simulink model "ARDroneHoverSim_backup_2026-11-11"  (R2025b)
settings: Solver=ode1  StartTime=0.0  StopTime=100  FixedStep=simDT  RelTol=1e-3  EnableMultiTasking=on
undefined symbols (not defined in the file or in its folder): FMS
libraries: ARBlocks x2
settings Model: Creator=Paul Freeman  LastModifiedBy=caio
settings SolverCC: AlgebraicLoopSolver=TrustRegion
settings DataIOCC: SaveFormat=Array  SignalLoggingSaveFormat=ModelDataLogs  SaveOutput=off  SignalLogging=off  ReturnWorkspaceOutputs=off
settings OptimizationCC: ExpressionDepthLimit=2147483647.0  LifeSpan=inf
settings DebuggingCC: UnderspecifiedInitializationDetection=Classic  MergeDetectMultiDrivingBlocksExec=none  SolverPrmCheckMsg=warning  MultiTaskDSMMsg=warning  MultiTaskCondExecSysMsg=none  FcnCallInpInsideContextMsg=warning  UnconnectedInputMsg=warning  UnconnectedOutputMsg=warning  UnconnectedLineMsg=warning  StateNameClashWarn=warning  SFUnexpectedBacktrackingDiag=warning  SFNoUnconditionalDefaultTransitionDiag=warning  SFExecutionAtInitializationDiag=none  ArithmeticOperatorsInVariantConditions=warning
settings HardwareCC: ProdBitPerPointer=32.0  ProdBitPerSizeT=32.0  ProdBitPerPtrDiffT=32.0  ProdLargestAtomicInteger=Long  ProdLargestAtomicFloat=Double  ProdEndianess=BigEndian  ProdWordSize=32.0  ProdHWDeviceType=Freescale->32-bit PowerPC
settings ModelReferenceCC: EnableRefExpFcnMdlSchedulingChecks=on  PropagateSignalLabelsOutOfModel=off
settings SFSimCC: SimUseLocalCustomCode=off  SimParseCustomCode=off  CustomCodeUndefinedFunction=UseInterfaceOnly
settings RTWCC: RTWUseLocalCustomCode=off  GPUComputeCapability=3.5
settings CodeAppCC: StateflowObjectComments=on
settings GRTTargetCC: TargetLangStandard=C89/C90 (ANSI)  CombineOutputUpdateFcns=off  GRTInterface=on
settings ConfigComp: CovMetricSettings=dw  CovSaveCumulativeToWorkspaceVar=on  CovSaveSingleToWorkspaceVar=on  CovExternalEMLEnable=off

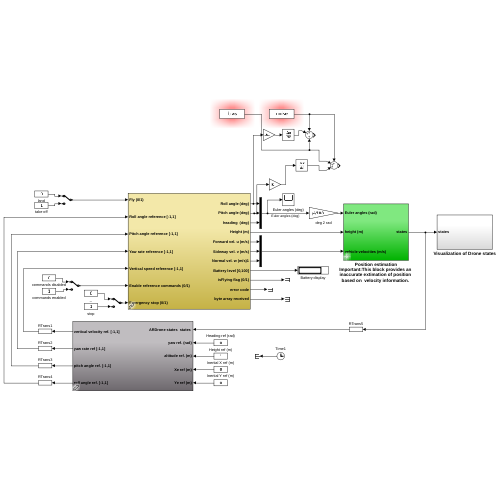
[thumbnail: Simulink's stored preview of the top-level diagram]
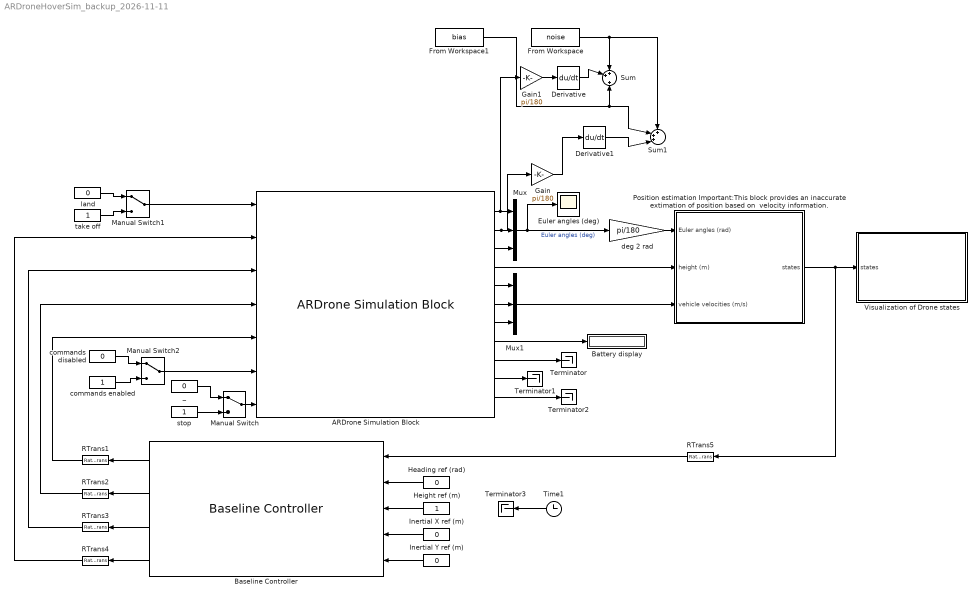
== system ARDroneHoverSim_backup_2026-11-11 ==
  ARDrone Simulation Block : ARBlocks/ARDrone Simulation Block  SystemSampleTime=-1  VariantActivationTime=update diagram  EmptyChoice=off  PassThrough=off  PassThroughVariantControl=(default)  EmptyChoiceVariantControl=(default)  AllowFlexibleInterface=on  Latency=0  AutoFrameSizeCalculation=off
  Baseline Controller : ARBlocks/Baseline Controller  SystemSampleTime=-1  VariantActivationTime=update diagram  EmptyChoice=off  PassThrough=off  PassThroughVariantControl=(default)  EmptyChoiceVariantControl=(default)  AllowFlexibleInterface=on  Latency=0  AutoFrameSizeCalculation=off
  Battery display : Display
  Derivative : Derivative
  Derivative1 : Derivative
  Euler angles (deg) : Scope
      settings: ActiveDisplayYMinimum=-22.5  ActiveDisplayYMaximum=22.5  DataLoggingMaxPoints=500000
  From Workspace : FromWorkspace  VariableName=noise
  From Workspace1 : FromWorkspace  VariableName=bias
  Gain : Gain  Gain=pi/180
  Gain1 : Gain  Gain=pi/180
  Heading ref (rad) : Constant  Value=0  SampleTime=FMS.Ts
  Height ref (m) : Constant  SampleTime=FMS.Ts
  Inertial X ref (m) : Constant  Value=0  SampleTime=FMS.Ts
  Inertial Y ref (m) : Constant  Value=0  SampleTime=FMS.Ts
  Manual Switch : ManualSwitch
  Manual Switch1 : ManualSwitch
  Manual Switch2 : ManualSwitch
  Mux : Mux  Inputs=3
  Mux1 : Mux  Inputs=3
  "Position estimation Important:This block provides an inaccurate extimation of position based on  velocity information. " : Subsystem  AncestorBlock=|
      | ARBlocks/Position estimation
      | Important:This block provides an 
      | inaccurate extimation of position 
      | based on  velocity information.
  RTrans{1..4} (4 alike) : RateTransition  OutPortSampleTime=simDT
  RTrans5 : RateTransition  OutPortSampleTime=FMS.Ts
  Sum : Sum  Inputs=++|+
  Sum1 : Sum  Inputs=+++|
  Terminator{,1..3} (4 alike) : Terminator
  Time1 : Clock
  Visualization of Drone states : Subsystem
  _ : Constant  Value=0
  commands disabled : Constant  Value=0
  commands enabled : Constant
  deg 2 rad : Gain  Gain=pi/180
  land : Constant  Value=0
  stop : Constant
  take off : Constant
  wires:
  _/1 -> Manual Switch/1
  stop/1 -> Manual Switch/2
  land/1 -> Manual Switch1/1
  take off/1 -> Manual Switch1/2
  commands disabled/1 -> Manual Switch2/1
  commands enabled/1 -> Manual Switch2/2
  Manual Switch1/1 -> ARDrone Simulation Block/1
  Manual Switch2/1 -> ARDrone Simulation Block/6
  Manual Switch/1 -> ARDrone Simulation Block/7
  ARDrone Simulation Block/1 -> Gain1/1, Mux/1
  ARDrone Simulation Block/2 -> Gain/1, Mux/2
  ARDrone Simulation Block/5 -> Mux1/1
  ARDrone Simulation Block/6 -> Mux1/2
  ARDrone Simulation Block/7 -> Mux1/3
  Mux/1 -> deg 2 rad/1, Euler angles (deg)/1  "Euler angles (deg)"
  ARDrone Simulation Block/8 -> Battery display/1
  Baseline Controller/1 -> RTrans1/1
  Baseline Controller/3 -> RTrans3/1
  "Position estimation Important:This block provides an inaccurate extimation of position based on  velocity information. "/1(states) -> RTrans5/1, Visualization of Drone states/1(states)
  deg 2 rad/1 -> "Position estimation Important:This block provides an inaccurate extimation of position based on  velocity information. "/1(Euler angles (rad))
  ARDrone Simulation Block/4 -> "Position estimation Important:This block provides an inaccurate extimation of position based on  velocity information. "/2(height (m))
  Mux1/1 -> "Position estimation Important:This block provides an inaccurate extimation of position based on  velocity information. "/3(vehicle velocities (m/s))
  Baseline Controller/2 -> RTrans2/1
  Baseline Controller/4 -> RTrans4/1
  ARDrone Simulation Block/3 -> Mux/3
  ARDrone Simulation Block/9 -> Terminator/1
  RTrans1/1 -> ARDrone Simulation Block/5
  RTrans2/1 -> ARDrone Simulation Block/4
  RTrans3/1 -> ARDrone Simulation Block/3
  RTrans4/1 -> ARDrone Simulation Block/2
  ARDrone Simulation Block/10 -> Terminator1/1
  ARDrone Simulation Block/11 -> Terminator2/1
  Time1/1 -> Terminator3/1
  Heading ref (rad)/1 -> Baseline Controller/2
  Height ref (m)/1 -> Baseline Controller/3
  Inertial X ref (m)/1 -> Baseline Controller/4
  Inertial Y ref (m)/1 -> Baseline Controller/5
  RTrans5/1 -> Baseline Controller/1
  Derivative/1 -> Sum/2
  From Workspace/1 -> Sum1/1, Sum/1
  From Workspace1/1 -> Sum1/2, Sum/3
  Derivative1/1 -> Sum1/3
  Gain/1 -> Derivative1/1
  Gain1/1 -> Derivative/1

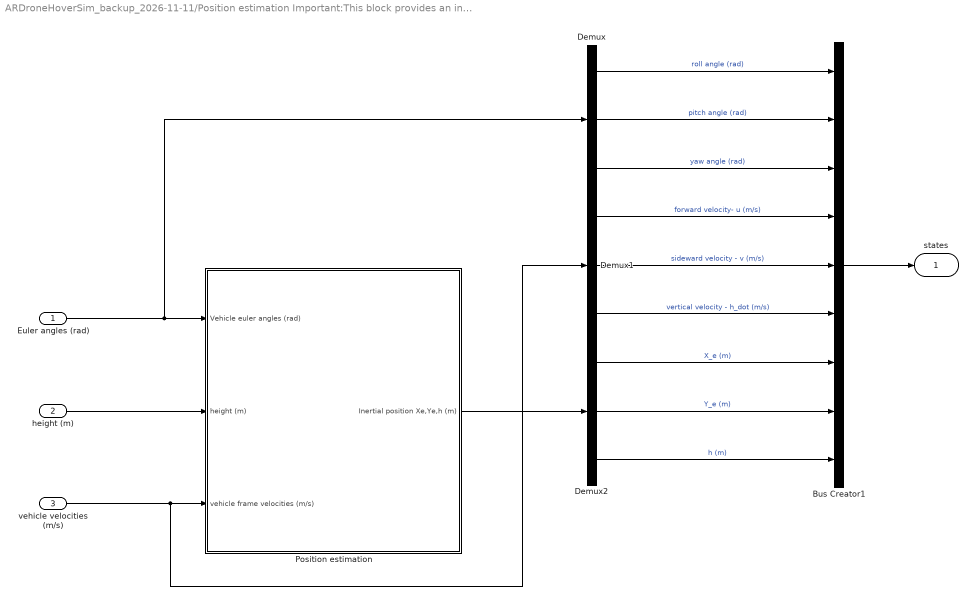
== system ARDroneHoverSim_backup_2026-11-11/Position estimation Important:This block provides an inaccurate extimation of position based on  velocity information.  ==
  Euler angles (rad) : Inport
  height (m) : Inport  Port=2
  vehicle velocities (m/s) : Inport  Port=3
  Bus Creator1 : BusCreator  Inputs=9
  Demux : Demux  Outputs=3
  Demux1 : Demux  Outputs=3
  Demux2 : Demux  Outputs=3
  Position estimation : Subsystem
  states : Outport
  wires:
  height (m)/1 -> Position estimation/2(height (m))
  Bus Creator1/1 -> states/1
  Demux2/3 -> Bus Creator1/9  "h (m)"
  Demux2/2 -> Bus Creator1/8  "Y_e (m)"
  Demux2/1 -> Bus Creator1/7  "X_e (m)"
  Demux1/3 -> Bus Creator1/6  "vertical velocity - h_dot (m/s)"
  Demux1/2 -> Bus Creator1/5  "sideward velocity - v (m/s)"
  Demux1/1 -> Bus Creator1/4  "forward velocity- u (m/s)"
  Demux/3 -> Bus Creator1/3  "yaw angle (rad)"
  Demux/2 -> Bus Creator1/2  "pitch angle (rad)"
  Demux/1 -> Bus Creator1/1  "roll angle (rad)"
  Position estimation/1(Inertial position Xe,Ye,h (m)) -> Demux2/1
  Euler angles (rad)/1 -> Demux/1, Position estimation/1(Vehicle euler angles (rad))
  vehicle velocities (m/s)/1 -> Position estimation/3(vehicle frame velocities (m/s)), Demux1/1

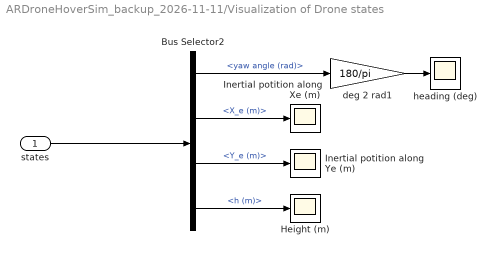
== system ARDroneHoverSim_backup_2026-11-11/Visualization of Drone states ==
  states : Inport
  Bus Selector2 : BusSelector  OutputSignals=yaw angle (rad),X_e (m),Y_e (m),h (m)
  Height (m) : Scope
      settings: ActiveDisplayYMinimum=-0.12689  ActiveDisplayYMaximum=1.0973  DataLoggingMaxPoints=500000  DataLoggingVariableName=ScopeData5
  Inertial potition along Xe (m) : Scope
      settings: ActiveDisplayYMinimum=-22.5  ActiveDisplayYMaximum=22.5  DataLoggingMaxPoints=500000  DataLoggingVariableName=ScopeData3
  Inertial potition along Ye (m) : Scope
      settings: ActiveDisplayYMinimum=-22.5  ActiveDisplayYMaximum=22.5  DataLoggingMaxPoints=500000  DataLoggingVariableName=ScopeData4
  deg 2 rad1 : Gain  Gain=180/pi
  heading (deg) : Scope
      settings: ActiveDisplayYMinimum=-22.5  ActiveDisplayYMaximum=22.5  DataLoggingMaxPoints=500000  DataLoggingVariableName=ScopeData2
  wires:
  states/1 -> Bus Selector2/1
  Bus Selector2/1 -> deg 2 rad1/1  "<yaw angle (rad)>"
  Bus Selector2/2 -> Inertial potition along Xe (m)/1  "<X_e (m)>"
  Bus Selector2/3 -> Inertial potition along Ye (m)/1  "<Y_e (m)>"
  Bus Selector2/4 -> Height (m)/1  "<h (m)>"
  deg 2 rad1/1 -> heading (deg)/1

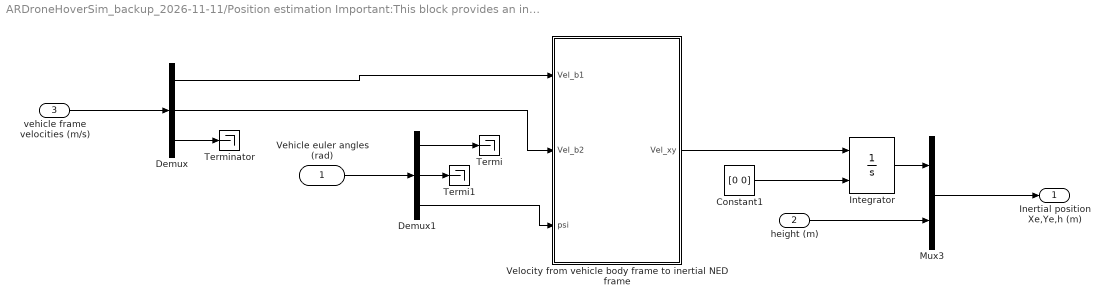
== system ARDroneHoverSim_backup_2026-11-11/Position estimation Important:This block provides an inaccurate extimation of position based on  velocity information. /Position estimation ==
  Vehicle euler angles (rad) : Inport
  height (m) : Inport  Port=2
  vehicle frame velocities (m/s) : Inport  Port=3
  Constant1 : Constant  Value=[0 0]
  Demux : Demux  Outputs=3
  Demux1 : Demux  Outputs=3
  Integrator : Integrator  InitialConditionSource=external
  Mux3 : Mux  Inputs=2
  Termi : Terminator
  Termi1 : Terminator
  Terminator : Terminator
  Velocity from vehicle body frame to inertial NED  frame : MATLAB Function  TreatAsAtomicUnit=on
  Inertial position Xe,Ye,h (m) : Outport
  wires:
  Mux3/1 -> Inertial position Xe,Ye,h (m)/1
  height (m)/1 -> Mux3/2
  Vehicle euler angles (rad)/1 -> Demux1/1
  vehicle frame velocities (m/s)/1 -> Demux/1
  Demux1/3 -> Velocity from vehicle body frame to inertial NED  frame/3(psi)
  Integrator/1 -> Mux3/1
  Constant1/1 -> Integrator/2
  Velocity from vehicle body frame to inertial NED  frame/1(Vel_xy) -> Integrator/1
  Demux1/2 -> Termi1/1
  Demux1/1 -> Termi/1
  Demux/1 -> Velocity from vehicle body frame to inertial NED  frame/1(Vel_b1)
  Demux/2 -> Velocity from vehicle body frame to inertial NED  frame/2(Vel_b2)
  Demux/3 -> Terminator/1

== matlab function ARDroneHoverSim_backup_2026-11-11/Position estimation Important:This block provides an inaccurate extimation of position based on  velocity information. /Position estimation/Velocity from vehicle body frame to inertial NED  frame ==
  data: Vel_b1 input; Vel_b2 input; Vel_xy output; psi input
function Vel_xy = fcn(Vel_b1, Vel_b2, psi)
%#codegen
T = [cos(psi) -sin(psi) ; sin(psi) cos(psi)] ; 
Vel_xy = T*[Vel_b1; Vel_b2];
